simulink model "fir_vtb_check"  (R2026a)
settings: Solver=FixedStepDiscrete  StopTime=400  FixedStep=1
model workspace (MAT data in the model file):
  b = [0.125 0.375 0.375 0.125]
libraries: vivadosimlib x1
settings Model: Creator=KoayXianCong  LastModifiedBy=KoayXianCong

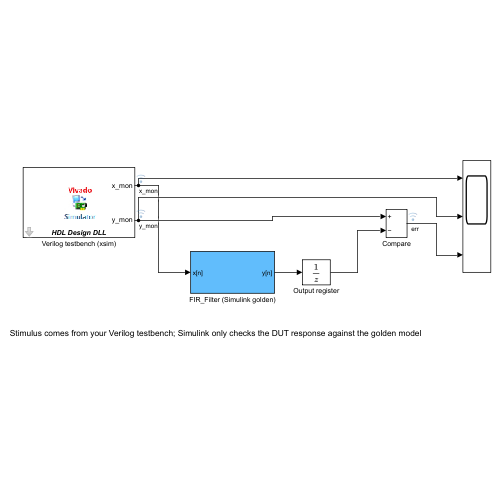
[thumbnail: Simulink's stored preview of the top-level diagram]
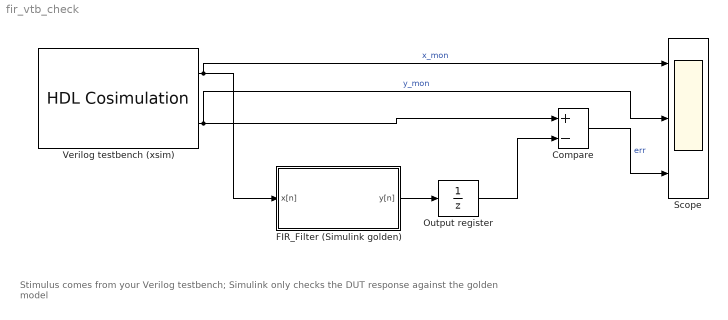
== system fir_vtb_check ==
  note: Stimulus comes from your Verilog testbench; Simulink only checks the DUT response against the golden model
  Compare : Sum  Inputs=+-
  FIR_Filter (Simulink golden) : Subsystem
  Output register : UnitDelay  SampleTime=-1
  Scope : Scope  NumInputPorts=3
      settings: TimeSpan=400
  Verilog testbench (xsim) : vivadosimlib/HDL Cosimulation  PortPaths=/tb_cosim_monitor/x_mon;/tb_cosim_monitor/y_mon;  PortModes=[2 2 ]  PortTimes=[1,1]  PortSigns=[1,1,]  PortFracLengths=[15,18]  PortWordLengths=[16,19]  PortHDLWordSizes=[16,19]  CommLocal=on  CommSharedMemory=off  CommPortNumber=0  CommShowInfo=on  ClockModes=[]  ClockTimes=[]  TimingMode=ns  TimingScaleFactor=10  idxCellArray={'UNUSED_VAR'}  CosimBypass=Full Simulation  AllowDirectFeedthrough=on  ProductName=EDA Simulator Link VS  RunAutoTimescale=off  PreRunTime=0  PreRunTimeUnit=ns
  wires:
  Verilog testbench (xsim)/1 -> FIR_Filter (Simulink golden)/1(x[n]), Scope/1  "x_mon"
  FIR_Filter (Simulink golden)/1(y[n]) -> Output register/1
  Verilog testbench (xsim)/2 -> Compare/1, Scope/2  "y_mon"
  Output register/1 -> Compare/2
  Compare/1 -> Scope/3  "err"

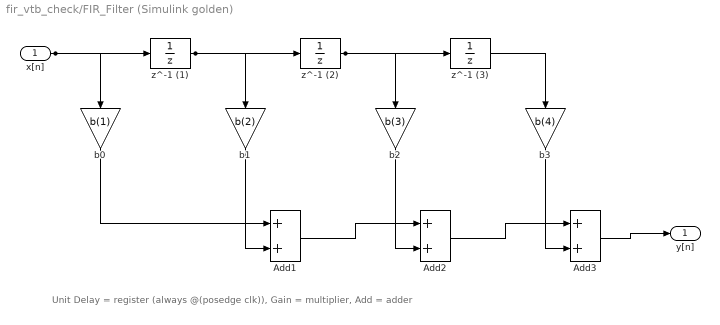
== system fir_vtb_check/FIR_Filter (Simulink golden) ==
  note: Unit Delay = register (always @(posedge clk)), Gain = multiplier, Add = adder
  x[n] : Inport
  Add1 : Sum  OutDataTypeStr=fixdt(1,19,18)
  Add2 : Sum  OutDataTypeStr=fixdt(1,19,18)
  Add3 : Sum  OutDataTypeStr=fixdt(1,19,18)
  b0 : Gain  Gain=b(1)  ParamDataTypeStr=fixdt(1,16,15)  OutDataTypeStr=fixdt(1,19,18)
  b1 : Gain  Gain=b(2)  ParamDataTypeStr=fixdt(1,16,15)  OutDataTypeStr=fixdt(1,19,18)
  b2 : Gain  Gain=b(3)  ParamDataTypeStr=fixdt(1,16,15)  OutDataTypeStr=fixdt(1,19,18)
  b3 : Gain  Gain=b(4)  ParamDataTypeStr=fixdt(1,16,15)  OutDataTypeStr=fixdt(1,19,18)
  z^-1 (1) : UnitDelay  SampleTime=-1
  z^-1 (2) : UnitDelay  SampleTime=-1
  z^-1 (3) : UnitDelay  SampleTime=-1
  y[n] : Outport
  wires:
  Add3/1 -> y[n]/1
  b3/1 -> Add3/2
  Add2/1 -> Add3/1
  b2/1 -> Add2/2
  Add1/1 -> Add2/1
  b1/1 -> Add1/2
  b0/1 -> Add1/1
  z^-1 (3)/1 -> b3/1
  z^-1 (2)/1 -> b2/1, z^-1 (3)/1
  z^-1 (1)/1 -> b1/1, z^-1 (2)/1
  x[n]/1 -> b0/1, z^-1 (1)/1
